simulink model "Powertrain_Comparison"  (R2024b)
settings: Solver=FixedStepDiscrete  StartTime=0.0  StopTime=3600  FixedStep=1  RelTol=1e-3
InitFcn:
  | try; sc=find_system(bdroot,'LookUnderMasks','all','FollowLinks','on','BlockType','Scope'); for k=1:numel(sc); c=get_param(sc{k},'ScopeConfiguration'); try; c.AxesScaling='Auto'; catch; end; try; nd=prod(c.LayoutDimensions); catch; nd=1; end; for d=1:nd; try; c.ActiveDisplay=d; catch; end; try; c.ShowLegend=true; catch; end; end; end; catch; end
(part 3 of 4)

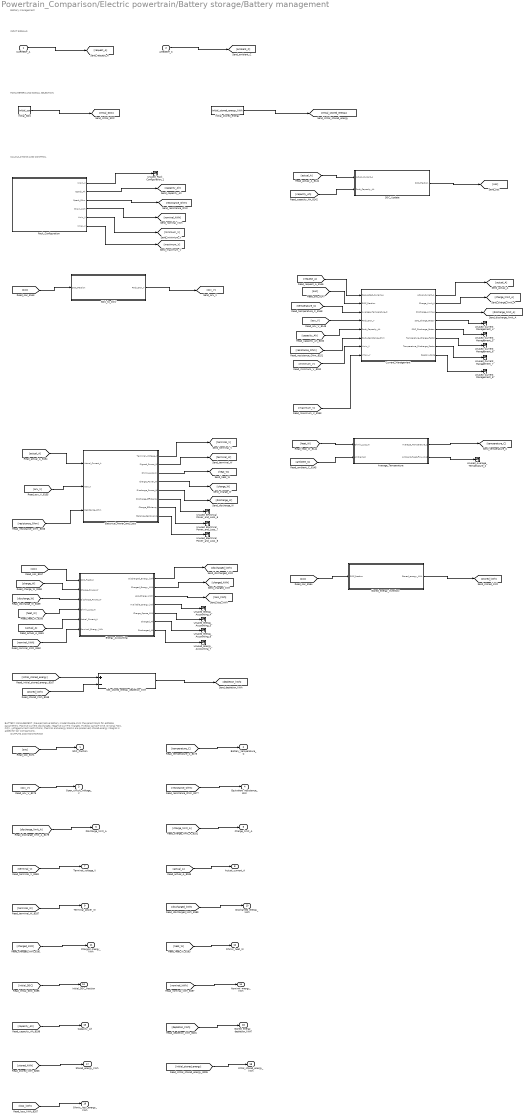
== system Powertrain_Comparison/Electric powertrain/Battery storage/Battery management ==
  note: BATTERY MANAGEMENT | Reused native battery model
      | Double-click the parent block for editable parameters. Positive current discharges; negative current charges. Fixed1s sample time.
      | Original SOC, OCV, voltage/current restrictions, thermal and energy blocks are preserved; stored-energy integral is added for fair comparisons.
  note: Battery management
  note: INPUT SIGNALS
  note: PARAMETERS AND SIGNAL SELECTION
  note: CALCULATIONS AND CONTROL
  note: OUTPUTS AND MONITORING
  CURRENT_A : Inport  PortDimensions=1
  AMBIENT_C : Inport  Port=2  PortDimensions=1
  Average_Temperature : Subsystem  Description=Equation 3.19 | One average thermal mass, I^2R heat, H(T-Ta) ambient transfer. No active cooling or hot-spot prediction.
  Current_Management : Subsystem  Description=Equations 3.20-3.29 | Most restrictive SOC, temperature, voltage and rated-current limits. A one-step SOC guard prevents numerical overshoot.
  Electrical_Power_and_Loss : Subsystem  Description=Equations 3.7-3.10 and 3.15-3.18 | Terminal voltage, signed power, I^2R loss and directional ohmic efficiency.
  Energy_Accounting : Subsystem  Description=Equations 3.11-3.14 and 3.16 | Separate energy-in, energy-out and loss accumulators; nominal-energy SOC-window estimates.
  Initial_SOC : Constant  Value=initial_soc
  Initial_stored_energy : Constant  Value=initial_stored_energy_kWh
  Net_stored_energy_depletion_kWh : Sum  Inputs=+-  InputSameDT=on  SaturateOnIntegerOverflow=on  OutDataTypeStr=Inherit: Same as first input
  Pack_Configuration : Subsystem  Description=Scaled balanced equivalent pack: Ns series groups and Np parallel cells.
  SOC_Update : Subsystem  Description=Equation 3.5 | Discrete coulomb counting. Positive current discharges. State is stored in a Unit Delay.
  SOC_to_OCV : Subsystem  Description=Equation 3.6 | Illustrative OCV lookup; replace with measured OCV data before experimental validation.
  Stored_energy_inventory : Subsystem
  Unused_Average_Temperature_2 : Terminator
  Unused_Current_Management_{4..8} (5 alike) : Terminator
  Unused_Electrical_Power_and_Loss_6 : Terminator
  Unused_Electrical_Power_and_Loss_7 : Terminator
  Unused_Electrical_Power_and_Loss_8 : Terminator
  Unused_Energy_Accounting_{4..7} (4 alike) : Terminator
  Unused_Pack_Configuration_1 : Terminator
  SOC_fraction : Outport  PortDimensions=1
  Battery_temperature_C : Outport  Port=2  PortDimensions=1
  Open_circuit_voltage_V : Outport  Port=3  PortDimensions=1
  Equivalent_resistance_ohm : Outport  Port=4  PortDimensions=1
  Discharge_limit_A : Outport  Port=5  PortDimensions=1
  Charge_limit_A : Outport  Port=6  PortDimensions=1
  Terminal_voltage_V : Outport  Port=7  PortDimensions=1
  Actual_current_A : Outport  Port=8  PortDimensions=1
  Terminal_power_W : Outport  Port=9  PortDimensions=1
  Discharged_energy_kWh : Outport  Port=10  PortDimensions=1
  Charged_energy_kWh : Outport  Port=11  PortDimensions=1
  Ohmic_heat_W : Outport  Port=12  PortDimensions=1
  Initial_SOC_fraction : Outport  Port=13  PortDimensions=1
  Nominal_energy_kWh : Outport  Port=14  PortDimensions=1
  Capacity_Ah : Outport  Port=15  PortDimensions=1
  Stored_energy_depletion_kWh : Outport  Port=16  PortDimensions=1
  Stored_energy_kWh : Outport  Port=17  PortDimensions=1
  Initial_stored_energy_kWh : Outport  Port=18  PortDimensions=1
  Ohmic_loss_energy_kWh : Outport  Port=19  PortDimensions=1
  wires:
  [maximum_V] -> Current_Management/8(Vmax_V)
  [actual_A] -> Actual_current_A/1
  [stored_kWh] -> Net_stored_energy_depletion_kWh/2
  Electrical_Power_and_Loss/1(Terminal_Voltage_V) -> [terminal_V]
  [ocv_V] -> Open_circuit_voltage_V/1
  CURRENT_A/1 -> [request_A]
  [charge_limit_A] -> Charge_limit_A/1
  [Initial_stored_energy] -> Net_stored_energy_depletion_kWh/1
  [discharged_kWh] -> Discharged_energy_kWh/1
  [soc] -> SOC_to_OCV/1(SOC_Fraction)
  [capacity_Ah] -> Current_Management/5(Pack_Capacity_Ah)
  [temperature_C] -> Battery_temperature_C/1
  [nominal_kWh] -> Nominal_energy_kWh/1
  SOC_Update/1(SOC_Fraction) -> [soc]
  [request_A] -> Current_Management/1(Requested_Current_A)
  [charged_kWh] -> Charged_energy_kWh/1
  Initial_stored_energy/1 -> [Initial_stored_energy]
  [ocv_V] -> Electrical_Power_and_Loss/2(OCV_V)
  Average_Temperature/2(Ambient_Heat_Flow_W_2) -> Unused_Average_Temperature_2/1
  [charge_W] -> Energy_Accounting/2(Charge_Power_W)
  [terminal_W] -> Terminal_power_W/1
  [heat_W] -> Ohmic_heat_W/1
  [actual_A] -> Electrical_Power_and_Loss/1(Actual_Current_A)
  [soc] -> Stored_energy_inventory/1(SOC_fraction)
  [actual_A] -> Energy_Accounting/5(Actual_Current_A)
  [soc] -> SOC_fraction/1
  [loss_kWh] -> Ohmic_loss_energy_kWh/1
  [resistance_Ohm] -> Current_Management/6(Pack_Resistance_Ohm)
  AMBIENT_C/1 -> [ambient_C]
  [depletion_kWh] -> Stored_energy_depletion_kWh/1
  [ocv_V] -> Current_Management/4(Pack_OCV_V)
  Average_Temperature/1(Average_Temperature_C) -> [temperature_C]
  [terminal_V] -> Terminal_voltage_V/1
  [capacity_Ah] -> Capacity_Ah/1
  [resistance_Ohm] -> Equivalent_resistance_ohm/1
  [discharge_limit_A] -> Discharge_limit_A/1
  [Initial_SOC] -> Initial_SOC_fraction/1
  [minimum_V] -> Current_Management/7(Vmin_V)
  [ambient_C] -> Average_Temperature/2(Ambient_C)
  [stored_kWh] -> Stored_energy_kWh/1
  [Initial_stored_energy] -> Initial_stored_energy_kWh/1
  [soc] -> Current_Management/2(SOC_Fraction)
  [heat_W] -> Average_Temperature/1(Ohmic_Loss_W)
  [actual_A] -> SOC_Update/1(Actual_Current_A)
  Electrical_Power_and_Loss/3(Ohmic_Loss_W) -> [heat_W]
  [heat_W] -> Energy_Accounting/4(Ohmic_Loss_W)
  [soc] -> Energy_Accounting/1(SOC_Fraction)
  [temperature_C] -> Current_Management/3(Average_Temperature_C)
  [nominal_kWh] -> Energy_Accounting/6(Nominal_Energy_kWh)
  [capacity_Ah] -> SOC_Update/2(Pack_Capacity_Ah)
  Pack_Configuration/1(Vnom_V) -> Unused_Pack_Configuration_1/1
  Pack_Configuration/2(Qpack_Ah) -> [capacity_Ah]
  Pack_Configuration/3(Rpack_Ohm) -> [resistance_Ohm]
  Pack_Configuration/4(Enom_kWh) -> [nominal_kWh]
  Pack_Configuration/5(Vmin_V) -> [minimum_V]
  Current_Management/1(Actual_Current_A) -> [actual_A]
  Pack_Configuration/6(Vmax_V) -> [maximum_V]
  [discharge_W] -> Energy_Accounting/3(Discharge_Power_W)
  [resistance_Ohm] -> Electrical_Power_and_Loss/3(Resistance_Ohm)
  Initial_SOC/1 -> [Initial_SOC]
  Net_stored_energy_depletion_kWh/1 -> [depletion_kWh]
  SOC_to_OCV/1(Pack_OCV_V) -> [ocv_V]
  Stored_energy_inventory/1(Stored_energy_kWh) -> [stored_kWh]
  Electrical_Power_and_Loss/2(Signed_Power_W) -> [terminal_W]
  Electrical_Power_and_Loss/4(Charge_Power_W) -> [charge_W]
  Electrical_Power_and_Loss/5(Discharge_Power_W) -> [discharge_W]
  Electrical_Power_and_Loss/6(Discharge_Efficiency) -> Unused_Electrical_Power_and_Loss_6/1
  Electrical_Power_and_Loss/7(Charge_Efficiency) -> Unused_Electrical_Power_and_Loss_7/1
  Electrical_Power_and_Loss/8(Balance_Residual_W) -> Unused_Electrical_Power_and_Loss_8/1
  Energy_Accounting/1(Discharged_Energy_kWh) -> [discharged_kWh]
  Energy_Accounting/2(Charged_Energy_kWh) -> [charged_kWh]
  Energy_Accounting/3(Loss_Energy_kWh) -> [loss_kWh]
  Energy_Accounting/4(Available_Energy_kWh) -> Unused_Energy_Accounting_4/1
  Energy_Accounting/5(Charge_Space_kWh) -> Unused_Energy_Accounting_5/1
  Energy_Accounting/6(Charged_Ah) -> Unused_Energy_Accounting_6/1
  Energy_Accounting/7(Discharged_Ah) -> Unused_Energy_Accounting_7/1
  Current_Management/2(Charge_Limit_A) -> [charge_limit_A]
  Current_Management/3(Discharge_Limit_A) -> [discharge_limit_A]
  Current_Management/4(SOC_Charge_Factor) -> Unused_Current_Management_4/1
  Current_Management/5(SOC_Discharge_Factor) -> Unused_Current_Management_5/1
  Current_Management/6(Temperature_Charge_Factor) -> Unused_Current_Management_6/1
  Current_Management/7(Temperature_Discharge_Factor) -> Unused_Current_Management_7/1
  Current_Management/8(Reason_Code) -> Unused_Current_Management_8/1

== system Powertrain_Comparison/Electric powertrain/Battery storage/Battery management/Average_Temperature ==
  note: Average Temperature
  note: Equation 3.19 | One average thermal mass, I^2R heat, H(T-Ta) ambient transfer. No active cooling or hot-spot prediction.
  note: OUTPUTS AND MONITORING
  Ohmic_Loss_W : Inport  PortDimensions=1
  Ambient_C : Inport  Port=2  PortDimensions=1
  Ambient_Conductance_W_K : Constant  Value=conductance_W_K
  Ambient_Heat_Flow_W : Product  Inputs=**  InputSameDT=on  RndMeth=Zero  SaturateOnIntegerOverflow=on  OutDataTypeStr=Inherit: Same as first input
  Net_Heat_J : Product  Inputs=**  InputSameDT=on  RndMeth=Zero  SaturateOnIntegerOverflow=on  OutDataTypeStr=Inherit: Same as first input
  Net_Heat_W : Sum  Inputs=+-  InputSameDT=on  SaturateOnIntegerOverflow=on  OutDataTypeStr=Inherit: Same as first input
  Pack_Mass_kg : Constant  Value=mass_kg
  Pack_Minus_Ambient_C : Sum  Inputs=+-  InputSameDT=on  SaturateOnIntegerOverflow=on  OutDataTypeStr=Inherit: Same as first input
  Sample_Time_s : Constant  Value=dt_s
  Specific_Heat_J_kgK : Constant  Value=cp_J_kgK
  Temperature_Increment : Product  Inputs=*/  InputSameDT=on  RndMeth=Zero  SaturateOnIntegerOverflow=on  OutDataTypeStr=Inherit: Same as first input
  Temperature_Next_Eq_3_19 : Sum  InputSameDT=on  SaturateOnIntegerOverflow=on  OutDataTypeStr=Inherit: Same as first input
  Temperature_State : UnitDelay  InitialCondition=initial_temp_C  SampleTime=dt_s
  Thermal_Capacity_J_K : Product  Inputs=**  InputSameDT=on  RndMeth=Zero  SaturateOnIntegerOverflow=on  OutDataTypeStr=Inherit: Same as first input
  Average_Temperature_C : Outport
  Ambient_Heat_Flow_W_2 : Outport  Port=2
  wires:
  Temperature_State/1 -> Temperature_Next_Eq_3_19/1, Pack_Minus_Ambient_C/1, Average_Temperature_C/1
  Ambient_Heat_Flow_W/1 -> Net_Heat_W/2, Ambient_Heat_Flow_W_2/1
  Sample_Time_s/1 -> Net_Heat_J/2
  Ohmic_Loss_W/1 -> Net_Heat_W/1
  Net_Heat_W/1 -> Net_Heat_J/1
  Pack_Minus_Ambient_C/1 -> Ambient_Heat_Flow_W/2
  Ambient_Conductance_W_K/1 -> Ambient_Heat_Flow_W/1
  Pack_Mass_kg/1 -> Thermal_Capacity_J_K/1
  Ambient_C/1 -> Pack_Minus_Ambient_C/2
  Specific_Heat_J_kgK/1 -> Thermal_Capacity_J_K/2
  Net_Heat_J/1 -> Temperature_Increment/1
  Thermal_Capacity_J_K/1 -> Temperature_Increment/2
  Temperature_Increment/1 -> Temperature_Next_Eq_3_19/2
  Temperature_Next_Eq_3_19/1 -> Temperature_State/1

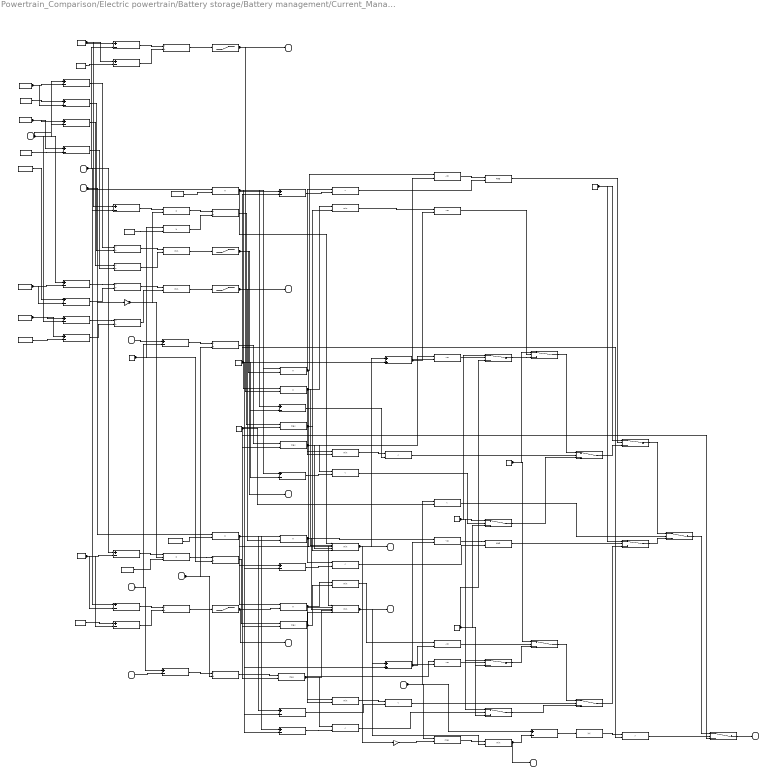
== system Powertrain_Comparison/Electric powertrain/Battery storage/Battery management/Current_Management ==
  note: Current Management
  note: Equations 3.20-3.29 | Most restrictive SOC, temperature, voltage and rated-current limits. A one-step SOC guard prevents
      | numerical overshoot.
  note: CALCULATIONS AND CONTROL
  Requested_Current_A : Inport  PortDimensions=1
  SOC_Fraction : Inport  Port=2  PortDimensions=1
  Average_Temperature_C : Inport  Port=3  PortDimensions=1
  Pack_OCV_V : Inport  Port=4  PortDimensions=1
  Pack_Capacity_Ah : Inport  Port=5  PortDimensions=1
  Pack_Resistance_Ohm : Inport  Port=6  PortDimensions=1
  Vmin_V : Inport  Port=7  PortDimensions=1
  Vmax_V : Inport  Port=8  PortDimensions=1
  Absolute_Current_Reduction : Abs
  Actual_Current_Eq_3_29 : MinMax  Inputs=2  InputSameDT=on  SaturateOnIntegerOverflow=on
  Charge_Above_Cold_Stop : Sum  Inputs=+-  InputSameDT=on  SaturateOnIntegerOverflow=on  OutDataTypeStr=Inherit: Same as first input
  Charge_Below_Hot_Stop : Sum  Inputs=+-  InputSameDT=on  SaturateOnIntegerOverflow=on  OutDataTypeStr=Inherit: Same as first input
  Charge_Below_Rated : Sum  Inputs=+-  InputSameDT=on  SaturateOnIntegerOverflow=on  OutDataTypeStr=Inherit: Same as first input
  Charge_Cold_Ramp : Product  Inputs=*/  InputSameDT=on  RndMeth=Zero  SaturateOnIntegerOverflow=on  OutDataTypeStr=Inherit: Same as first input
  Charge_Cold_Transition : Sum  Inputs=+-  InputSameDT=on  SaturateOnIntegerOverflow=on  OutDataTypeStr=Inherit: Same as first input
  Charge_Current_Rating_C : Constant  Value=charge_rate_C
  Charge_Efficiency : Constant  Value=eta_charge
  Charge_Fallback_Voltage : Switch  Threshold=0.5
  Charge_Full_Current_Lower_C : Constant  Value=charge_T2_C
  Charge_Full_Current_Upper_C : Constant  Value=charge_T3_C
  Charge_Headroom_C : Product  Inputs=**  InputSameDT=on  RndMeth=Zero  SaturateOnIntegerOverflow=on  OutDataTypeStr=Inherit: Same as first input
  Charge_Headroom_SOC : Sum  Inputs=+-  InputSameDT=on  SaturateOnIntegerOverflow=on  OutDataTypeStr=Inherit: Same as first input
  Charge_Hot_Ramp : Product  Inputs=*/  InputSameDT=on  RndMeth=Zero  SaturateOnIntegerOverflow=on  OutDataTypeStr=Inherit: Same as first input
  Charge_Hot_Transition : Sum  Inputs=+-  InputSameDT=on  SaturateOnIntegerOverflow=on  OutDataTypeStr=Inherit: Same as first input
  Charge_Limit_Tolerance : Sum  InputSameDT=on  SaturateOnIntegerOverflow=on  OutDataTypeStr=Inherit: Same as first input
  Charge_Lower_Stop_C : Constant  Value=charge_T1_C
  Charge_Rated_Minus_Eps : Sum  Inputs=+-  InputSameDT=on  SaturateOnIntegerOverflow=on  OutDataTypeStr=Inherit: Same as first input
  Charge_Request : RelationalOperator  Operator=<  OutDataTypeStr='double'
  Charge_SOC_Combined : MinMax  Inputs=2  InputSameDT=on  SaturateOnIntegerOverflow=on
  Charge_SOC_Is_Min : RelationalOperator  Operator=<=  OutDataTypeStr='double'
  Charge_SOC_Limits : MinMax  Inputs=2  InputSameDT=on  SaturateOnIntegerOverflow=on
  Charge_SOC_Margin : Product  Inputs=*/  InputSameDT=on  RndMeth=Zero  SaturateOnIntegerOverflow=on  OutDataTypeStr=Inherit: Same as first input
  Charge_SOC_Not_Active : Switch  Threshold=0.5
  Charge_SOC_Reason : Switch  Threshold=0.5
  Charge_SOC_Reduced : RelationalOperator  Operator=<  OutDataTypeStr='double'
  Charge_Step_Cap : Product  Inputs=*/  InputSameDT=on  RndMeth=Zero  SaturateOnIntegerOverflow=on  OutDataTypeStr=Inherit: Same as first input
  Charge_Step_Efficiency : Product  Inputs=**  InputSameDT=on  RndMeth=Zero  SaturateOnIntegerOverflow=on  OutDataTypeStr=Inherit: Same as first input
  Charge_Step_Headroom_A : MinMax  Function=max  Inputs=2  InputSameDT=on  SaturateOnIntegerOverflow=on
  Charge_Taper_SOC : Constant  Value=soc_taper
  Charge_Taper_Width : Sum  Inputs=+-  InputSameDT=on  SaturateOnIntegerOverflow=on  OutDataTypeStr=Inherit: Same as first input
  Charge_Temperature_Factor_Eq_3_22 : Saturate  UpperLimit=1  LowerLimit=0
  Charge_Temperature_Ramps : MinMax  Inputs=2  InputSameDT=on  SaturateOnIntegerOverflow=on
  Charge_Temperature_Reason : Switch  Threshold=0.5
  Charge_Thermal_Is_Active : Logic  Description=Logical AND of the thermal-limit predicates. The output controls the reason-code selector; this is not numeric power multiplication.  AllPortsSameDT=off  OutDataTypeStr=boolean
  Charge_Thermal_Is_Min : RelationalOperator  Operator=<=  OutDataTypeStr='double'
  Charge_Thermal_Rated_Eps : Sum  Inputs=+-  InputSameDT=on  SaturateOnIntegerOverflow=on  OutDataTypeStr=Inherit: Same as first input
  Charge_Thermal_Reduced : RelationalOperator  Operator=<  OutDataTypeStr='double'
  Charge_Upper_Stop_C : Constant  Value=charge_T4_C
  Charge_Voltage_Below_Rated : RelationalOperator  Operator=<  OutDataTypeStr='double'
  Charge_Voltage_Is_Min : RelationalOperator  Operator=<=  OutDataTypeStr='double'
  Charge_Voltage_Margin_A : Product  Inputs=*/  InputSameDT=on  RndMeth=Zero  SaturateOnIntegerOverflow=on  OutDataTypeStr=Inherit: Same as first input
  Charge_Voltage_Reason : Switch  Threshold=0.5
  Current_Reduction : Sum  Inputs=+-  InputSameDT=on  SaturateOnIntegerOverflow=on  OutDataTypeStr=Inherit: Same as first input
  Discharge_Above_Cold_Stop : Sum  Inputs=+-  InputSameDT=on  SaturateOnIntegerOverflow=on  OutDataTypeStr=Inherit: Same as first input
  Discharge_Below_Hot_Stop : Sum  Inputs=+-  InputSameDT=on  SaturateOnIntegerOverflow=on  OutDataTypeStr=Inherit: Same as first input
  Discharge_Below_Rated : Sum  Inputs=+-  InputSameDT=on  SaturateOnIntegerOverflow=on  OutDataTypeStr=Inherit: Same as first input
  Discharge_Cold_Ramp : Product  Inputs=*/  InputSameDT=on  RndMeth=Zero  SaturateOnIntegerOverflow=on  OutDataTypeStr=Inherit: Same as first input
  Discharge_Cold_Transition : Sum  Inputs=+-  InputSameDT=on  SaturateOnIntegerOverflow=on  OutDataTypeStr=Inherit: Same as first input
  Discharge_Current_Rating_C : Constant  Value=discharge_rate_C
  Discharge_Efficiency : Constant  Value=eta_discharge
  Discharge_Fallback_Voltage : Switch  Threshold=0.5
  Discharge_Full_Current_Lower_C : Constant  Value=discharge_T2_C
  Discharge_Full_Current_Upper_C : Constant  Value=discharge_T3_C
  Discharge_Headroom_C : Product  Inputs=***  InputSameDT=on  RndMeth=Zero  SaturateOnIntegerOverflow=on  OutDataTypeStr=Inherit: Same as first input
  Discharge_Headroom_SOC : Sum  Inputs=+-  InputSameDT=on  SaturateOnIntegerOverflow=on  OutDataTypeStr=Inherit: Same as first input
  Discharge_Hot_Ramp : Product  Inputs=*/  InputSameDT=on  RndMeth=Zero  SaturateOnIntegerOverflow=on  OutDataTypeStr=Inherit: Same as first input
  Discharge_Hot_Transition : Sum  Inputs=+-  InputSameDT=on  SaturateOnIntegerOverflow=on  OutDataTypeStr=Inherit: Same as first input
  Discharge_Limit_Tolerance : Sum  InputSameDT=on  SaturateOnIntegerOverflow=on  OutDataTypeStr=Inherit: Same as first input
  Discharge_Lower_Stop_C : Constant  Value=discharge_T1_C
  Discharge_Rated_Minus_Eps : Sum  Inputs=+-  InputSameDT=on  SaturateOnIntegerOverflow=on  OutDataTypeStr=Inherit: Same as first input
  Discharge_Reserve_SOC : Constant  Value=soc_reserve
  Discharge_SOC_Combined : MinMax  Inputs=2  InputSameDT=on  SaturateOnIntegerOverflow=on
  Discharge_SOC_Is_Min : RelationalOperator  Operator=<=  OutDataTypeStr='double'
  Discharge_SOC_Limits : MinMax  Inputs=2  InputSameDT=on  SaturateOnIntegerOverflow=on
  Discharge_SOC_Margin : Product  Inputs=*/  InputSameDT=on  RndMeth=Zero  SaturateOnIntegerOverflow=on  OutDataTypeStr=Inherit: Same as first input
  Discharge_SOC_Not_Active : Switch  Threshold=0.5
  Discharge_SOC_Reason : Switch  Threshold=0.5
  Discharge_SOC_Reduced : RelationalOperator  Operator=<  OutDataTypeStr='double'
  Discharge_Step_Cap : Product  Inputs=*/  InputSameDT=on  RndMeth=Zero  SaturateOnIntegerOverflow=on  OutDataTypeStr=Inherit: Same as first input
  Discharge_Step_Headroom_A : MinMax  Function=max  Inputs=2  InputSameDT=on  SaturateOnIntegerOverflow=on
  Discharge_Taper_Width : Sum  Inputs=+-  InputSameDT=on  SaturateOnIntegerOverflow=on  OutDataTypeStr=Inherit: Same as first input
  Discharge_Temperature_Factor_Eq_3_22 : Saturate  UpperLimit=1  LowerLimit=0
  Discharge_Temperature_Ramps : MinMax  Inputs=2  InputSameDT=on  SaturateOnIntegerOverflow=on
  Discharge_Temperature_Reason : Switch  Threshold=0.5
  Discharge_Thermal_Is_Active : Logic  Description=Logical AND of the thermal-limit predicates. The output controls the reason-code selector; this is not numeric power multiplication.  AllPortsSameDT=off  OutDataTypeStr=boolean
  Discharge_Thermal_Is_Min : RelationalOperator  Operator=<=  OutDataTypeStr='double'
  Discharge_Thermal_Rated_Eps : Sum  Inputs=+-  InputSameDT=on  SaturateOnIntegerOverflow=on  OutDataTypeStr=Inherit: Same as first input
  Discharge_Thermal_Reduced : RelationalOperator  Operator=<  OutDataTypeStr='double'
  Discharge_Upper_Stop_C : Constant  Value=discharge_T4_C
  Discharge_Voltage_Below_Rated : RelationalOperator  Operator=<  OutDataTypeStr='double'
  Discharge_Voltage_Is_Min : RelationalOperator  Operator=<=  OutDataTypeStr='double'
  Discharge_Voltage_Margin_A : Product  Inputs=*/  InputSameDT=on  RndMeth=Zero  SaturateOnIntegerOverflow=on  OutDataTypeStr=Inherit: Same as first input
  Discharge_Voltage_Reason : Switch  Threshold=0.5
  Limiting_Reason_Code : Switch  Threshold=0.5
  Lower_Charge_Clamp : MinMax  Function=max  Inputs=2  InputSameDT=on  SaturateOnIntegerOverflow=on
  Lower_SOC_Reserve : Sum  Inputs=+-  InputSameDT=on  SaturateOnIntegerOverflow=on  OutDataTypeStr=Inherit: Same as first input
  Lower_Voltage_Margin : Sum  Inputs=+-  InputSameDT=on  SaturateOnIntegerOverflow=on  OutDataTypeStr=Inherit: Same as first input
  Maximum_Charge_Current_Eq_3_27 : MinMax  Inputs=5  InputSameDT=on  SaturateOnIntegerOverflow=on
  Maximum_Discharge_Current_Eq_3_28 : MinMax  Inputs=5  InputSameDT=on  SaturateOnIntegerOverflow=on
  Maximum_SOC : Constant  Value=soc_max
  Minimum_SOC : Constant  Value=soc_min
  Negative_Charge_Limit : Gain  Gain=-1  SaturateOnIntegerOverflow=on  OutDataTypeStr=Inherit: Same as input  ParamDataTypeStr=Inherit: Same as input
  Pack_Charge_Coulombs : Gain  Gain=3600  SaturateOnIntegerOverflow=on  OutDataTypeStr=Inherit: Same as input  ParamDataTypeStr=Inherit: Same as input
  Rated_Charge_Current_A : Product  Inputs=**  InputSameDT=on  RndMeth=Zero  SaturateOnIntegerOverflow=on  OutDataTypeStr=Inherit: Same as first input
  Rated_Discharge_Current_A : Product  Inputs=**  InputSameDT=on  RndMeth=Zero  SaturateOnIntegerOverflow=on  OutDataTypeStr=Inherit: Same as first input
  Reason_Rated : Constant
  Reason_SOC : Constant  Value=2
  Reason_Temperature : Constant  Value=3
  Reason_Voltage : Constant  Value=4
  Request_Is_Limited : RelationalOperator  Operator=>  OutDataTypeStr='double'
  SOC_Charge_Factor_Eq_3_20 : Saturate  UpperLimit=1  LowerLimit=0
  SOC_Charge_Limit_A : Product  Inputs=**  InputSameDT=on  RndMeth=Zero  SaturateOnIntegerOverflow=on  OutDataTypeStr=Inherit: Same as first input
  SOC_Discharge_Factor_Eq_3_21 : Saturate  UpperLimit=1  LowerLimit=0
  SOC_Discharge_Limit_A : Product  Inputs=**  InputSameDT=on  RndMeth=Zero  SaturateOnIntegerOverflow=on  OutDataTypeStr=Inherit: Same as first input
  Selected_Direction_Reason : Switch  Threshold=0.5
  Step_Time_s : Constant  Value=dt_s
  Thermal_Charge_Limit_A : Product  Inputs=**  InputSameDT=on  RndMeth=Zero  SaturateOnIntegerOverflow=on  OutDataTypeStr=Inherit: Same as first input
  Thermal_Discharge_Limit_A : Product  Inputs=**  InputSameDT=on  RndMeth=Zero  SaturateOnIntegerOverflow=on  OutDataTypeStr=Inherit: Same as first input
  Tolerance : Constant  Value=1e-08
  Upper_SOC_Space : Sum  Inputs=+-  InputSameDT=on  SaturateOnIntegerOverflow=on  OutDataTypeStr=Inherit: Same as first input
  Upper_Voltage_Margin : Sum  Inputs=+-  InputSameDT=on  SaturateOnIntegerOverflow=on  OutDataTypeStr=Inherit: Same as first input
  Voltage_Charge_Limit_Eq_3_25 : MinMax  Function=max  Inputs=2  InputSameDT=on  SaturateOnIntegerOverflow=on
  Voltage_Discharge_Limit_Eq_3_26 : MinMax  Function=max  Inputs=2  InputSameDT=on  SaturateOnIntegerOverflow=on
  Zero : Constant  Value=0
  Actual_Current_A : Outport
  Charge_Limit_A : Outport  Port=2
  Discharge_Limit_A : Outport  Port=3
  SOC_Charge_Factor : Outport  Port=4
  SOC_Discharge_Factor : Outport  Port=5
  Temperature_Charge_Factor : Outport  Port=6
  Temperature_Discharge_Factor : Outport  Port=7
  Reason_Code : Outport  Port=8
  wires:
  Current_Reduction/1 -> Absolute_Current_Reduction/1
  Lower_Charge_Clamp/1 -> Actual_Current_Eq_3_29/1
  Maximum_Discharge_Current_Eq_3_28/1 -> Actual_Current_Eq_3_29/2, Discharge_Limit_Tolerance/1, Discharge_Limit_A/1
  Average_Temperature_C/1 -> Charge_Above_Cold_Stop/1, Charge_Below_Hot_Stop/2, Discharge_Above_Cold_Stop/1, Discharge_Below_Hot_Stop/2
  Charge_Lower_Stop_C/1 -> Charge_Above_Cold_Stop/2, Charge_Cold_Transition/2
  Charge_Upper_Stop_C/1 -> Charge_Below_Hot_Stop/1, Charge_Hot_Transition/1
  Rated_Charge_Current_A/1 -> Charge_Below_Rated/1, Charge_Rated_Minus_Eps/1, Charge_Thermal_Rated_Eps/1, Maximum_Charge_Current_Eq_3_27/1, SOC_Charge_Limit_A/1, Thermal_Charge_Limit_A/1
  Tolerance/1 -> Charge_Below_Rated/2, Charge_Limit_Tolerance/2, Charge_Rated_Minus_Eps/2, Charge_Thermal_Rated_Eps/2, Discharge_Below_Rated/2, Discharge_Limit_Tolerance/2, Discharge_Rated_Minus_Eps/2, Discharge_Thermal_Rated_Eps/2, Request_Is_Limited/2
  Charge_Above_Cold_Stop/1 -> Charge_Cold_Ramp/1
  Charge_Cold_Transition/1 -> Charge_Cold_Ramp/2
  Charge_Full_Current_Lower_C/1 -> Charge_Cold_Transition/1
  Reason_Voltage/1 -> Charge_Fallback_Voltage/1, Charge_Voltage_Reason/1, Discharge_Fallback_Voltage/1, Discharge_Voltage_Reason/1
  Charge_Voltage_Below_Rated/1 -> Charge_Fallback_Voltage/2
  Reason_Rated/1 -> Charge_Fallback_Voltage/3, Charge_Voltage_Reason/3, Discharge_Fallback_Voltage/3, Discharge_Voltage_Reason/3
  Charge_Headroom_SOC/1 -> Charge_Headroom_C/1
  Pack_Charge_Coulombs/1 -> Charge_Headroom_C/2, Discharge_Headroom_C/2
  Maximum_SOC/1 -> Charge_Headroom_SOC/1, Charge_Taper_Width/1, Upper_SOC_Space/1
  SOC_Fraction/1 -> Charge_Headroom_SOC/2, Discharge_Headroom_SOC/1, Lower_SOC_Reserve/1, Upper_SOC_Space/2
  Charge_Below_Hot_Stop/1 -> Charge_Hot_Ramp/1
  Charge_Hot_Transition/1 -> Charge_Hot_Ramp/2
  Charge_Full_Current_Upper_C/1 -> Charge_Hot_Transition/2
  Maximum_Charge_Current_Eq_3_27/1 -> Charge_Limit_Tolerance/1, Negative_Charge_Limit/1, Charge_Limit_A/1
  Requested_Current_A/1 -> Charge_Request/1, Current_Reduction/1, Lower_Charge_Clamp/1
  Zero/1 -> Charge_Request/2, Charge_Step_Headroom_A/2, Discharge_Step_Headroom_A/2, Limiting_Reason_Code/3, Voltage_Charge_Limit_Eq_3_25/2, Voltage_Discharge_Limit_Eq_3_26/2
  SOC_Charge_Limit_A/1 -> Charge_SOC_Combined/1, Charge_SOC_Limits/1, Maximum_Charge_Current_Eq_3_27/2
  Charge_Step_Headroom_A/1 -> Charge_SOC_Combined/2, Charge_SOC_Limits/2, Maximum_Charge_Current_Eq_3_27/5
  Charge_SOC_Combined/1 -> Charge_SOC_Is_Min/1
  Charge_Limit_Tolerance/1 -> Charge_SOC_Is_Min/2, Charge_Thermal_Is_Min/2, Charge_Voltage_Is_Min/2
  Upper_SOC_Space/1 -> Charge_SOC_Margin/1
  Charge_Taper_Width/1 -> Charge_SOC_Margin/2
  Charge_SOC_Reason/1 -> Charge_SOC_Not_Active/1
  Charge_SOC_Reduced/1 -> Charge_SOC_Not_Active/2
  Charge_Fallback_Voltage/1 -> Charge_SOC_Not_Active/3
  Reason_SOC/1 -> Charge_SOC_Reason/1, Discharge_SOC_Reason/1
  Charge_SOC_Is_Min/1 -> Charge_SOC_Reason/2
  Charge_Voltage_Reason/1 -> Charge_SOC_Reason/3
  Charge_SOC_Limits/1 -> Charge_SOC_Reduced/1
  Charge_Below_Rated/1 -> Charge_SOC_Reduced/2
  Charge_Headroom_C/1 -> Charge_Step_Cap/1
  Charge_Step_Efficiency/1 -> Charge_Step_Cap/2
  Step_Time_s/1 -> Charge_Step_Efficiency/1, Discharge_Step_Cap/2
  Charge_Efficiency/1 -> Charge_Step_Efficiency/2
  Charge_Step_Cap/1 -> Charge_Step_Headroom_A/1
  Charge_Taper_SOC/1 -> Charge_Taper_Width/2
  Charge_Temperature_Ramps/1 -> Charge_Temperature_Factor_Eq_3_22/1
  Charge_Cold_Ramp/1 -> Charge_Temperature_Ramps/1
  Charge_Hot_Ramp/1 -> Charge_Temperature_Ramps/2
  Reason_Temperature/1 -> Charge_Temperature_Reason/1, Discharge_Temperature_Reason/1
  Charge_Thermal_Is_Active/1 -> Charge_Temperature_Reason/2
  Charge_SOC_Not_Active/1 -> Charge_Temperature_Reason/3
  Charge_Thermal_Is_Min/1 -> Charge_Thermal_Is_Active/1
  Charge_Thermal_Reduced/1 -> Charge_Thermal_Is_Active/2
  Thermal_Charge_Limit_A/1 -> Charge_Thermal_Is_Min/1, Charge_Thermal_Reduced/1, Maximum_Charge_Current_Eq_3_27/3
  Charge_Thermal_Rated_Eps/1 -> Charge_Thermal_Reduced/2
  Voltage_Charge_Limit_Eq_3_25/1 -> Charge_Voltage_Below_Rated/1, Charge_Voltage_Is_Min/1, Maximum_Charge_Current_Eq_3_27/4
  Charge_Rated_Minus_Eps/1 -> Charge_Voltage_Below_Rated/2
  Upper_Voltage_Margin/1 -> Charge_Voltage_Margin_A/1
  Pack_Resistance_Ohm/1 -> Charge_Voltage_Margin_A/2, Discharge_Voltage_Margin_A/2
  Charge_Voltage_Is_Min/1 -> Charge_Voltage_Reason/2
  Actual_Current_Eq_3_29/1 -> Current_Reduction/2, Actual_Current_A/1
  Discharge_Lower_Stop_C/1 -> Discharge_Above_Cold_Stop/2, Discharge_Cold_Transition/2
  Discharge_Upper_Stop_C/1 -> Discharge_Below_Hot_Stop/1, Discharge_Hot_Transition/1
  Rated_Discharge_Current_A/1 -> Discharge_Below_Rated/1, Discharge_Rated_Minus_Eps/1, Discharge_Thermal_Rated_Eps/1, Maximum_Discharge_Current_Eq_3_28/1, SOC_Discharge_Limit_A/1, Thermal_Discharge_Limit_A/1
  Discharge_Above_Cold_Stop/1 -> Discharge_Cold_Ramp/1
  Discharge_Cold_Transition/1 -> Discharge_Cold_Ramp/2
  Discharge_Full_Current_Lower_C/1 -> Discharge_Cold_Transition/1
  Discharge_Voltage_Below_Rated/1 -> Discharge_Fallback_Voltage/2
  Discharge_Headroom_SOC/1 -> Discharge_Headroom_C/1
  Discharge_Efficiency/1 -> Discharge_Headroom_C/3
  Minimum_SOC/1 -> Discharge_Headroom_SOC/2, Discharge_Taper_Width/2, Lower_SOC_Reserve/2
  Discharge_Below_Hot_Stop/1 -> Discharge_Hot_Ramp/1
  Discharge_Hot_Transition/1 -> Discharge_Hot_Ramp/2
  Discharge_Full_Current_Upper_C/1 -> Discharge_Hot_Transition/2
  SOC_Discharge_Limit_A/1 -> Discharge_SOC_Combined/1, Discharge_SOC_Limits/1, Maximum_Discharge_Current_Eq_3_28/2
  Discharge_Step_Headroom_A/1 -> Discharge_SOC_Combined/2, Discharge_SOC_Limits/2, Maximum_Discharge_Current_Eq_3_28/5
  Discharge_SOC_Combined/1 -> Discharge_SOC_Is_Min/1
  Discharge_Limit_Tolerance/1 -> Discharge_SOC_Is_Min/2, Discharge_Thermal_Is_Min/2, Discharge_Voltage_Is_Min/2
  Lower_SOC_Reserve/1 -> Discharge_SOC_Margin/1
  Discharge_Taper_Width/1 -> Discharge_SOC_Margin/2
  Discharge_SOC_Reason/1 -> Discharge_SOC_Not_Active/1
  Discharge_SOC_Reduced/1 -> Discharge_SOC_Not_Active/2
  Discharge_Fallback_Voltage/1 -> Discharge_SOC_Not_Active/3
  Discharge_SOC_Is_Min/1 -> Discharge_SOC_Reason/2
  Discharge_Voltage_Reason/1 -> Discharge_SOC_Reason/3
  Discharge_SOC_Limits/1 -> Discharge_SOC_Reduced/1
  Discharge_Below_Rated/1 -> Discharge_SOC_Reduced/2
  Discharge_Headroom_C/1 -> Discharge_Step_Cap/1
  Discharge_Step_Cap/1 -> Discharge_Step_Headroom_A/1
  Discharge_Reserve_SOC/1 -> Discharge_Taper_Width/1
  Discharge_Temperature_Ramps/1 -> Discharge_Temperature_Factor_Eq_3_22/1
  Discharge_Cold_Ramp/1 -> Discharge_Temperature_Ramps/1
  Discharge_Hot_Ramp/1 -> Discharge_Temperature_Ramps/2
  Discharge_Thermal_Is_Active/1 -> Discharge_Temperature_Reason/2
  Discharge_SOC_Not_Active/1 -> Discharge_Temperature_Reason/3
  Discharge_Thermal_Is_Min/1 -> Discharge_Thermal_Is_Active/1
  Discharge_Thermal_Reduced/1 -> Discharge_Thermal_Is_Active/2
  Thermal_Discharge_Limit_A/1 -> Discharge_Thermal_Is_Min/1, Discharge_Thermal_Reduced/1, Maximum_Discharge_Current_Eq_3_28/3
  Discharge_Thermal_Rated_Eps/1 -> Discharge_Thermal_Reduced/2
  Voltage_Discharge_Limit_Eq_3_26/1 -> Discharge_Voltage_Below_Rated/1, Discharge_Voltage_Is_Min/1, Maximum_Discharge_Current_Eq_3_28/4
  Discharge_Rated_Minus_Eps/1 -> Discharge_Voltage_Below_Rated/2
  Lower_Voltage_Margin/1 -> Discharge_Voltage_Margin_A/1
  Discharge_Voltage_Is_Min/1 -> Discharge_Voltage_Reason/2
  Selected_Direction_Reason/1 -> Limiting_Reason_Code/1
  Request_Is_Limited/1 -> Limiting_Reason_Code/2
  Negative_Charge_Limit/1 -> Lower_Charge_Clamp/2
  Pack_OCV_V/1 -> Lower_Voltage_Margin/1, Upper_Voltage_Margin/2
  Vmin_V/1 -> Lower_Voltage_Margin/2
  Pack_Capacity_Ah/1 -> Pack_Charge_Coulombs/1, Rated_Charge_Current_A/1, Rated_Discharge_Current_A/1
  Charge_Current_Rating_C/1 -> Rated_Charge_Current_A/2
  Discharge_Current_Rating_C/1 -> Rated_Discharge_Current_A/2
  Absolute_Current_Reduction/1 -> Request_Is_Limited/1
  Charge_SOC_Margin/1 -> SOC_Charge_Factor_Eq_3_20/1
  SOC_Charge_Factor_Eq_3_20/1 -> SOC_Charge_Limit_A/2, SOC_Charge_Factor/1
  Discharge_SOC_Margin/1 -> SOC_Discharge_Factor_Eq_3_21/1
  SOC_Discharge_Factor_Eq_3_21/1 -> SOC_Discharge_Limit_A/2, SOC_Discharge_Factor/1
  Charge_Temperature_Reason/1 -> Selected_Direction_Reason/1
  Charge_Request/1 -> Selected_Direction_Reason/2
  Discharge_Temperature_Reason/1 -> Selected_Direction_Reason/3
  Charge_Temperature_Factor_Eq_3_22/1 -> Thermal_Charge_Limit_A/2, Temperature_Charge_Factor/1
  Discharge_Temperature_Factor_Eq_3_22/1 -> Thermal_Discharge_Limit_A/2, Temperature_Discharge_Factor/1
  Vmax_V/1 -> Upper_Voltage_Margin/1
  Charge_Voltage_Margin_A/1 -> Voltage_Charge_Limit_Eq_3_25/1
  Discharge_Voltage_Margin_A/1 -> Voltage_Discharge_Limit_Eq_3_26/1
  Limiting_Reason_Code/1 -> Reason_Code/1

== system Powertrain_Comparison/Electric powertrain/Battery storage/Battery management/Electrical_Power_and_Loss ==
  note: Electrical Power and Loss
  note: Equations 3.7-3.10 and 3.15-3.18 | Terminal voltage, signed power, I^2R loss and directional ohmic efficiency.
  note: CALCULATIONS AND CONTROL
  Actual_Current_A : Inport  PortDimensions=1
  OCV_V : Inport  Port=2  PortDimensions=1
  Resistance_Ohm : Inport  Port=3  PortDimensions=1
  Charge_Active : RelationalOperator  Operator=>  OutDataTypeStr='double'
  Charge_After_Loss : Sum  Inputs=+-  InputSameDT=on  SaturateOnIntegerOverflow=on  OutDataTypeStr=Inherit: Same as first input
  Charge_Efficiency_Eq_3_18 : Switch  Threshold=0.5
  Charge_Efficiency_Ratio : Product  Inputs=*/  InputSameDT=on  RndMeth=Zero  SaturateOnIntegerOverflow=on  OutDataTypeStr=Inherit: Same as first input
  Charge_Power_Eq_3_10 : MinMax  Function=max  Inputs=2  InputSameDT=on  SaturateOnIntegerOverflow=on
  Charge_Safe_Denominator : MinMax  Function=max  Inputs=2  InputSameDT=on  SaturateOnIntegerOverflow=on
  Chemical_Discharge_Power : Sum  InputSameDT=on  SaturateOnIntegerOverflow=on  OutDataTypeStr=Inherit: Same as first input
  Discharge_Active : RelationalOperator  Operator=>  OutDataTypeStr='double'
  Discharge_Efficiency_Eq_3_17 : Switch  Threshold=0.5
  Discharge_Power_Eq_3_9 : MinMax  Function=max  Inputs=2  InputSameDT=on  SaturateOnIntegerOverflow=on
  Discharge_Safe_Denominator : MinMax  Function=max  Inputs=2  InputSameDT=on  SaturateOnIntegerOverflow=on
  Efficiency_Not_Applicable : Constant  Value=-1
  IR_Voltage_Drop : Product  Inputs=**  InputSameDT=on  RndMeth=Zero  SaturateOnIntegerOverflow=on  OutDataTypeStr=Inherit: Same as first input
  Negative_Terminal_Power : Gain  Gain=-1  SaturateOnIntegerOverflow=on  OutDataTypeStr=Inherit: Same as input  ParamDataTypeStr=Inherit: Same as input
  OCV_Power_W : Product  Inputs=**  InputSameDT=on  RndMeth=Zero  SaturateOnIntegerOverflow=on  OutDataTypeStr=Inherit: Same as first input
  Ohmic_Loss_Eq_3_15 : Product  Inputs=***  InputSameDT=on  RndMeth=Zero  SaturateOnIntegerOverflow=on  OutDataTypeStr=Inherit: Same as first input
  Power_Balance_Residual_W : Sum  Inputs=+--  InputSameDT=on  SaturateOnIntegerOverflow=on  OutDataTypeStr=Inherit: Same as first input
  Power_Tolerance_W : Constant  Value=1e-09
  Signed_Power_Eq_3_8 : Product  Inputs=**  InputSameDT=on  RndMeth=Zero  SaturateOnIntegerOverflow=on  OutDataTypeStr=Inherit: Same as first input
  Terminal_Voltage_Eq_3_7 : Sum  Inputs=+-  InputSameDT=on  SaturateOnIntegerOverflow=on  OutDataTypeStr=Inherit: Same as first input
  Useful_Charge_Fraction : MinMax  Function=max  Inputs=2  InputSameDT=on  SaturateOnIntegerOverflow=on
  Useful_Discharge_Fraction : Product  Inputs=*/  InputSameDT=on  RndMeth=Zero  SaturateOnIntegerOverflow=on  OutDataTypeStr=Inherit: Same as first input
  Zero : Constant  Value=0
  Terminal_Voltage_V : Outport
  Signed_Power_W : Outport  Port=2
  Ohmic_Loss_W : Outport  Port=3
  Charge_Power_W : Outport  Port=4
  Discharge_Power_W : Outport  Port=5
  Discharge_Efficiency : Outport  Port=6
  Charge_Efficiency : Outport  Port=7
  Balance_Residual_W : Outport  Port=8
  wires:
  Charge_Power_Eq_3_10/1 -> Charge_Active/1, Charge_After_Loss/1, Charge_Safe_Denominator/1, Charge_Power_W/1
  Power_Tolerance_W/1 -> Charge_Active/2, Charge_Safe_Denominator/2, Discharge_Active/2, Discharge_Safe_Denominator/2
  Ohmic_Loss_Eq_3_15/1 -> Charge_After_Loss/2, Chemical_Discharge_Power/2, Power_Balance_Residual_W/3, Ohmic_Loss_W/1
  Useful_Charge_Fraction/1 -> Charge_Efficiency_Eq_3_18/1
  Charge_Active/1 -> Charge_Efficiency_Eq_3_18/2
  Efficiency_Not_Applicable/1 -> Charge_Efficiency_Eq_3_18/3, Discharge_Efficiency_Eq_3_17/3
  Charge_After_Loss/1 -> Charge_Efficiency_Ratio/1
  Charge_Safe_Denominator/1 -> Charge_Efficiency_Ratio/2
  Negative_Terminal_Power/1 -> Charge_Power_Eq_3_10/1
  Zero/1 -> Charge_Power_Eq_3_10/2, Discharge_Power_Eq_3_9/2, Useful_Charge_Fraction/2
  Discharge_Power_Eq_3_9/1 -> Chemical_Discharge_Power/1, Discharge_Active/1, Useful_Discharge_Fraction/1, Discharge_Power_W/1
  Useful_Discharge_Fraction/1 -> Discharge_Efficiency_Eq_3_17/1
  Discharge_Active/1 -> Discharge_Efficiency_Eq_3_17/2
  Signed_Power_Eq_3_8/1 -> Discharge_Power_Eq_3_9/1, Negative_Terminal_Power/1, Power_Balance_Residual_W/2, Signed_Power_W/1
  Chemical_Discharge_Power/1 -> Discharge_Safe_Denominator/1
  Actual_Current_A/1 -> IR_Voltage_Drop/1, OCV_Power_W/2, Ohmic_Loss_Eq_3_15/1, Ohmic_Loss_Eq_3_15/2, Signed_Power_Eq_3_8/2
  Resistance_Ohm/1 -> IR_Voltage_Drop/2, Ohmic_Loss_Eq_3_15/3
  OCV_V/1 -> OCV_Power_W/1, Terminal_Voltage_Eq_3_7/1
  OCV_Power_W/1 -> Power_Balance_Residual_W/1
  Terminal_Voltage_Eq_3_7/1 -> Signed_Power_Eq_3_8/1, Terminal_Voltage_V/1
  IR_Voltage_Drop/1 -> Terminal_Voltage_Eq_3_7/2
  Charge_Efficiency_Ratio/1 -> Useful_Charge_Fraction/1
  Discharge_Safe_Denominator/1 -> Useful_Discharge_Fraction/2
  Discharge_Efficiency_Eq_3_17/1 -> Discharge_Efficiency/1
  Charge_Efficiency_Eq_3_18/1 -> Charge_Efficiency/1
  Power_Balance_Residual_W/1 -> Balance_Residual_W/1

== system Powertrain_Comparison/Electric powertrain/Battery storage/Battery management/Energy_Accounting ==
  note: Energy Accounting
  note: Equations 3.11-3.14 and 3.16 | Separate energy-in, energy-out and loss accumulators; nominal-energy SOC-window estimates.
  note: OUTPUTS AND MONITORING
  SOC_Fraction : Inport  PortDimensions=1
  Charge_Power_W : Inport  Port=2  PortDimensions=1
  Discharge_Power_W : Inport  Port=3  PortDimensions=1
  Ohmic_Loss_W : Inport  Port=4  PortDimensions=1
  Actual_Current_A : Inport  Port=5  PortDimensions=1
  Nominal_Energy_kWh : Inport  Port=6  PortDimensions=1
  Available_Energy_Eq_3_13 : Product  Inputs=**  InputSameDT=on  RndMeth=Zero  SaturateOnIntegerOverflow=on  OutDataTypeStr=Inherit: Same as first input
  Charge_In_Ah_Increment : Gain  Gain=dt_s/3600  SaturateOnIntegerOverflow=on  OutDataTypeStr=Inherit: Same as input  ParamDataTypeStr=Inherit: Same as input
  Charge_In_Ah_Next : Sum  InputSameDT=on  SaturateOnIntegerOverflow=on  OutDataTypeStr=Inherit: Same as first input
  Charge_In_Ah_State : UnitDelay  SampleTime=dt_s
  Charge_Out_Ah_Increment : Gain  Gain=dt_s/3600  SaturateOnIntegerOverflow=on  OutDataTypeStr=Inherit: Same as input  ParamDataTypeStr=Inherit: Same as input
  Charge_Out_Ah_Next : Sum  InputSameDT=on  SaturateOnIntegerOverflow=on  OutDataTypeStr=Inherit: Same as first input
  Charge_Out_Ah_State : UnitDelay  SampleTime=dt_s
  Charge_SOC_Window : Sum  Inputs=+-  InputSameDT=on  SaturateOnIntegerOverflow=on  OutDataTypeStr=Inherit: Same as first input
  Charge_Space_Eq_3_14 : Product  Inputs=**  InputSameDT=on  RndMeth=Zero  SaturateOnIntegerOverflow=on  OutDataTypeStr=Inherit: Same as first input
  Charged_Energy_kWh_Increment : Gain  Gain=dt_s/3.6e6  SaturateOnIntegerOverflow=on  OutDataTypeStr=Inherit: Same as input  ParamDataTypeStr=Inherit: Same as input
  Charged_Energy_kWh_Next : Sum  InputSameDT=on  SaturateOnIntegerOverflow=on  OutDataTypeStr=Inherit: Same as first input
  Charged_Energy_kWh_State : UnitDelay  SampleTime=dt_s
  Charging_Current_Magnitude : MinMax  Function=max  Inputs=2  InputSameDT=on  SaturateOnIntegerOverflow=on
  Discharge_Current_Magnitude : MinMax  Function=max  Inputs=2  InputSameDT=on  SaturateOnIntegerOverflow=on
  Discharge_SOC_Window : Sum  Inputs=+-  InputSameDT=on  SaturateOnIntegerOverflow=on  OutDataTypeStr=Inherit: Same as first input
  Discharged_Energy_kWh_Increment : Gain  Gain=dt_s/3.6e6  SaturateOnIntegerOverflow=on  OutDataTypeStr=Inherit: Same as input  ParamDataTypeStr=Inherit: Same as input
  Discharged_Energy_kWh_Next : Sum  InputSameDT=on  SaturateOnIntegerOverflow=on  OutDataTypeStr=Inherit: Same as first input
  Discharged_Energy_kWh_State : UnitDelay  SampleTime=dt_s
  Loss_Energy_kWh_Increment : Gain  Gain=dt_s/3.6e6  SaturateOnIntegerOverflow=on  OutDataTypeStr=Inherit: Same as input  ParamDataTypeStr=Inherit: Same as input
  Loss_Energy_kWh_Next : Sum  InputSameDT=on  SaturateOnIntegerOverflow=on  OutDataTypeStr=Inherit: Same as first input
  Loss_Energy_kWh_State : UnitDelay  SampleTime=dt_s
  Maximum_SOC : Constant  Value=soc_max
  Minimum_SOC : Constant  Value=soc_min
  Negative_Current : Gain  Gain=-1  SaturateOnIntegerOverflow=on  OutDataTypeStr=Inherit: Same as input  ParamDataTypeStr=Inherit: Same as input
  SOC_Above_Reserve : MinMax  Function=max  Inputs=2  InputSameDT=on  SaturateOnIntegerOverflow=on
  SOC_Below_Upper_Limit : MinMax  Function=max  Inputs=2  InputSameDT=on  SaturateOnIntegerOverflow=on
  Zero : Constant  Value=0
  Discharged_Energy_kWh : Outport
  Charged_Energy_kWh : Outport  Port=2
  Loss_Energy_kWh : Outport  Port=3
  Available_Energy_kWh : Outport  Port=4
  Charge_Space_kWh : Outport  Port=5
  Charged_Ah : Outport  Port=6
  Discharged_Ah : Outport  Port=7
  wires:
  Ohmic_Loss_W/1 -> Loss_Energy_kWh_Increment/1
  Charge_SOC_Window/1 -> SOC_Below_Upper_Limit/1
  Charge_Out_Ah_State/1 -> Charge_Out_Ah_Next/1, Discharged_Ah/1
  SOC_Below_Upper_Limit/1 -> Charge_Space_Eq_3_14/2
  Charge_Power_W/1 -> Charged_Energy_kWh_Increment/1
  Maximum_SOC/1 -> Charge_SOC_Window/1
  SOC_Fraction/1 -> Charge_SOC_Window/2, Discharge_SOC_Window/1
  Actual_Current_A/1 -> Negative_Current/1, Discharge_Current_Magnitude/1
  Discharge_Power_W/1 -> Discharged_Energy_kWh_Increment/1
  Charge_In_Ah_State/1 -> Charged_Ah/1, Charge_In_Ah_Next/1
  Minimum_SOC/1 -> Discharge_SOC_Window/2
  Charged_Energy_kWh_Increment/1 -> Charged_Energy_kWh_Next/2
  Loss_Energy_kWh_Increment/1 -> Loss_Energy_kWh_Next/2
  Zero/1 -> Discharge_Current_Magnitude/2, SOC_Above_Reserve/2, Charging_Current_Magnitude/2, SOC_Below_Upper_Limit/2
  Charged_Energy_kWh_State/1 -> Charged_Energy_kWh_Next/1, Charged_Energy_kWh/1
  Loss_Energy_kWh_State/1 -> Loss_Energy_kWh_Next/1, Loss_Energy_kWh/1
  Discharge_SOC_Window/1 -> SOC_Above_Reserve/1
  Discharged_Energy_kWh_Increment/1 -> Discharged_Energy_kWh_Next/2
  Charge_Space_Eq_3_14/1 -> Charge_Space_kWh/1
  Nominal_Energy_kWh/1 -> Available_Energy_Eq_3_13/1, Charge_Space_Eq_3_14/1
  Discharged_Energy_kWh_State/1 -> Discharged_Energy_kWh_Next/1, Discharged_Energy_kWh/1
  Charge_Out_Ah_Increment/1 -> Charge_Out_Ah_Next/2
  Negative_Current/1 -> Charging_Current_Magnitude/1
  Discharge_Current_Magnitude/1 -> Charge_Out_Ah_Increment/1
  Charge_In_Ah_Increment/1 -> Charge_In_Ah_Next/2
  Charged_Energy_kWh_Next/1 -> Charged_Energy_kWh_State/1
  Loss_Energy_kWh_Next/1 -> Loss_Energy_kWh_State/1
  SOC_Above_Reserve/1 -> Available_Energy_Eq_3_13/2
  Discharged_Energy_kWh_Next/1 -> Discharged_Energy_kWh_State/1
  Charging_Current_Magnitude/1 -> Charge_In_Ah_Increment/1
  Available_Energy_Eq_3_13/1 -> Available_Energy_kWh/1
  Charge_Out_Ah_Next/1 -> Charge_Out_Ah_State/1
  Charge_In_Ah_Next/1 -> Charge_In_Ah_State/1

== system Powertrain_Comparison/Electric powertrain/Battery storage/Battery management/Pack_Configuration ==
  note: Pack Configuration
  note: Equations 3.1-3.4 | 96s24p | eight 12s24p modules | balanced equivalent pack.
  note: CALCULATIONS AND CONTROL
  Cell_Capacity_Ah : Constant  Value=cell_capacity_Ah
  Cell_DC_Resistance_Ohm : Constant  Value=cell_resistance_ohm
  Cell_Maximum_V : Constant  Value=cell_max_V
  Cell_Minimum_V : Constant  Value=cell_min_V
  Cell_Nominal_V : Constant  Value=cell_nominal_V
  Maximum_Pack_V : Product  Inputs=**  InputSameDT=on  RndMeth=Zero  SaturateOnIntegerOverflow=on  OutDataTypeStr=Inherit: Same as first input
  Minimum_Pack_V : Product  Inputs=**  InputSameDT=on  RndMeth=Zero  SaturateOnIntegerOverflow=on  OutDataTypeStr=Inherit: Same as first input
  Nominal_Energy_kWh_Eq_3_3 : Gain  Gain=0.001  SaturateOnIntegerOverflow=on  OutDataTypeStr=Inherit: Same as input  ParamDataTypeStr=Inherit: Same as input
  Ns_over_Np : Product  Inputs=*/  InputSameDT=on  RndMeth=Zero  SaturateOnIntegerOverflow=on  OutDataTypeStr=Inherit: Same as first input
  Pack_Capacity_Ah_Eq_3_2 : Product  Inputs=**  InputSameDT=on  RndMeth=Zero  SaturateOnIntegerOverflow=on  OutDataTypeStr=Inherit: Same as first input
  Pack_Nominal_V_Eq_3_1 : Product  Inputs=**  InputSameDT=on  RndMeth=Zero  SaturateOnIntegerOverflow=on  OutDataTypeStr=Inherit: Same as first input
  Pack_Resistance_Eq_3_4 : Product  Inputs=**  InputSameDT=on  RndMeth=Zero  SaturateOnIntegerOverflow=on  OutDataTypeStr=Inherit: Same as first input
  Parallel_Cells_Np : Constant  Value=np
  Series_Groups_Ns : Constant  Value=ns
  Volt_Ah : Product  Inputs=**  InputSameDT=on  RndMeth=Zero  SaturateOnIntegerOverflow=on  OutDataTypeStr=Inherit: Same as first input
  Vnom_V : Outport
  Qpack_Ah : Outport  Port=2
  Rpack_Ohm : Outport  Port=3
  Enom_kWh : Outport  Port=4
  Vmin_V : Outport  Port=5
  Vmax_V : Outport  Port=6
  wires:
  Cell_Maximum_V/1 -> Maximum_Pack_V/2
  Cell_Capacity_Ah/1 -> Pack_Capacity_Ah_Eq_3_2/2
  Cell_Nominal_V/1 -> Pack_Nominal_V_Eq_3_1/2
  Parallel_Cells_Np/1 -> Pack_Capacity_Ah_Eq_3_2/1, Ns_over_Np/2
  Pack_Capacity_Ah_Eq_3_2/1 -> Volt_Ah/2, Qpack_Ah/1
  Pack_Nominal_V_Eq_3_1/1 -> Vnom_V/1, Volt_Ah/1
  Series_Groups_Ns/1 -> Ns_over_Np/1, Pack_Nominal_V_Eq_3_1/1, Minimum_Pack_V/1, Maximum_Pack_V/1
  Cell_Minimum_V/1 -> Minimum_Pack_V/2
  Ns_over_Np/1 -> Pack_Resistance_Eq_3_4/1
  Cell_DC_Resistance_Ohm/1 -> Pack_Resistance_Eq_3_4/2
  Maximum_Pack_V/1 -> Vmax_V/1
  Minimum_Pack_V/1 -> Vmin_V/1
  Volt_Ah/1 -> Nominal_Energy_kWh_Eq_3_3/1
  Pack_Resistance_Eq_3_4/1 -> Rpack_Ohm/1
  Nominal_Energy_kWh_Eq_3_3/1 -> Enom_kWh/1

== system Powertrain_Comparison/Electric powertrain/Battery storage/Battery management/SOC_Update ==
  note: SOC Update
  note: Equation 3.5 | Discrete coulomb counting. Positive current discharges. State is stored in a Unit Delay.
  note: OUTPUTS AND MONITORING
  Actual_Current_A : Inport  PortDimensions=1
  Pack_Capacity_Ah : Inport  Port=2  PortDimensions=1
  Ampere_Seconds_to_SOC : Gain  Gain=-dt_s/3600  SaturateOnIntegerOverflow=on  OutDataTypeStr=Inherit: Same as input  ParamDataTypeStr=Inherit: Same as input
  Capacity_Normalisation : Product  Inputs=*/  InputSameDT=on  RndMeth=Zero  SaturateOnIntegerOverflow=on  OutDataTypeStr=Inherit: Same as first input
  Charge_Coulombic_Efficiency : Constant  Value=eta_charge
  Directional_Efficiency : Switch  Threshold=0.5
  Discharge_Coulombic_Efficiency : Constant  Value=eta_discharge
  Discharging : RelationalOperator  OutDataTypeStr='double'
  Effective_Current : Product  Inputs=**  InputSameDT=on  RndMeth=Zero  SaturateOnIntegerOverflow=on  OutDataTypeStr=Inherit: Same as first input
  One : Constant
  Reciprocal_Discharge_Efficiency : Product  Inputs=*/  InputSameDT=on  RndMeth=Zero  SaturateOnIntegerOverflow=on  OutDataTypeStr=Inherit: Same as first input
  SOC_Boundaries : Saturate  UpperLimit=soc_max  LowerLimit=soc_min
  SOC_Next_Eq_3_5 : Sum  InputSameDT=on  SaturateOnIntegerOverflow=on  OutDataTypeStr=Inherit: Same as first input
  SOC_State : UnitDelay  InitialCondition=initial_soc  SampleTime=dt_s
  Zero : Constant  Value=0
  SOC_Fraction : Outport
  wires:
  Reciprocal_Discharge_Efficiency/1 -> Directional_Efficiency/1
  Zero/1 -> Discharging/2
  One/1 -> Reciprocal_Discharge_Efficiency/1
  Discharging/1 -> Directional_Efficiency/2
  Discharge_Coulombic_Efficiency/1 -> Reciprocal_Discharge_Efficiency/2
  Directional_Efficiency/1 -> Effective_Current/1
  Actual_Current_A/1 -> Effective_Current/2, Discharging/1
  Charge_Coulombic_Efficiency/1 -> Directional_Efficiency/3
  Effective_Current/1 -> Capacity_Normalisation/1
  Pack_Capacity_Ah/1 -> Capacity_Normalisation/2
  Capacity_Normalisation/1 -> Ampere_Seconds_to_SOC/1
  Ampere_Seconds_to_SOC/1 -> SOC_Next_Eq_3_5/2
  SOC_State/1 -> SOC_Next_Eq_3_5/1, SOC_Fraction/1
  SOC_Next_Eq_3_5/1 -> SOC_Boundaries/1
  SOC_Boundaries/1 -> SOC_State/1

== system Powertrain_Comparison/Electric powertrain/Battery storage/Battery management/SOC_to_OCV ==
  note: SOC to OCV
  note: Equation 3.6 | Illustrative OCV lookup; replace with measured OCV data before experimental validation.
  note: OUTPUTS AND MONITORING
  SOC_Fraction : Inport  PortDimensions=1
  Cell_OCV_Lookup : Lookup_n-D  Description=Illustrative monotonic OCV curve, NOT measured P42A OCV data. Replace before experimental validation.  NumberOfTableDimensions=1  BreakpointsForDimension1=ocv_soc  Table=ocv_cell_V  ExtrapMethod=Clip
  Pack_OCV_Eq_3_6 : Gain  Gain=ns  SaturateOnIntegerOverflow=on  OutDataTypeStr=Inherit: Same as input  ParamDataTypeStr=Inherit: Same as input
  Pack_OCV_V : Outport
  wires:
  SOC_Fraction/1 -> Cell_OCV_Lookup/1
  Cell_OCV_Lookup/1 -> Pack_OCV_Eq_3_6/1
  Pack_OCV_Eq_3_6/1 -> Pack_OCV_V/1
